simulink model "Model_LQR_Ideal"  (R2025a)
settings: Solver=ode4  StartTime=0.0  StopTime=inf  FixedStep=0.0001  RelTol=1e-3
InitFcn:
  | addpath('functions');
model workspace: external: MATLAB File D:\OneDrive - University of Bristol\2025-2026\grp-major_project - General\LQR\furuta-inverted-pendulum-LQR\init_LQR.m (data not in the file)
values from neighbouring files (symbols this model uses):
  I_1 = in2(:,4)    [furuta_single_A_B_matrices.m]    (also in furuta_single_state_derivative.m = in4(:,4); init_LQR.m = 0.00011)
  I_arm = in2(:,2)    [furuta_single_A_B_matrices.m]    (also in furuta_single_state_derivative.m = in4(:,2); init_LQR.m = 0.000739)
  init_S = [0; 0; 0.26; 0]    [init_LQR.m]
  K = lqr(A, B, Q, R)    [init_LQR.m]
  L_1 = 0.14    [init_LQR.m]    (also in playback_animation_single.m = out.plotData.L_1.Data(1))
  L_arm = in2(:,1)    [furuta_single_A_B_matrices.m]    (also in furuta_single_state_derivative.m = in4(:,1); init_LQR.m = 0.1475; playback_animation_single.m = out.plotData.L_arm.Data(1))
  lcom_1 = in2(:,3)    [furuta_single_A_B_matrices.m]    (also in furuta_single_state_derivative.m = in4(:,3); init_LQR.m = 0.051; playback_animation_single.m = out.plotData.lcom_1.Data(1))
  m_1 = in2(:,5)    [furuta_single_A_B_matrices.m]    (also in furuta_single_state_derivative.m = in4(:,5); init_LQR.m = 0.054)
settings Model: PacingRate=0.010000  Creator=Esther  LastModifiedBy=Hankin

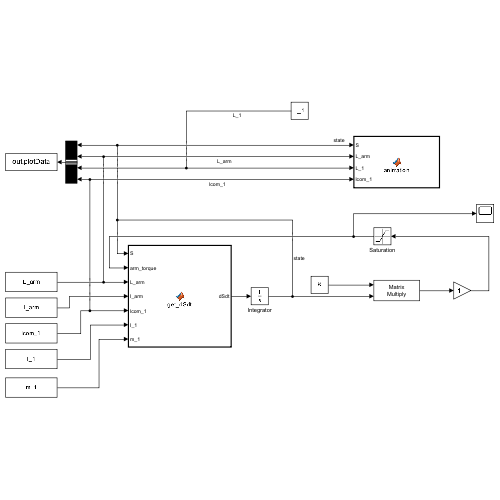
[thumbnail: Simulink's stored preview of the top-level diagram]
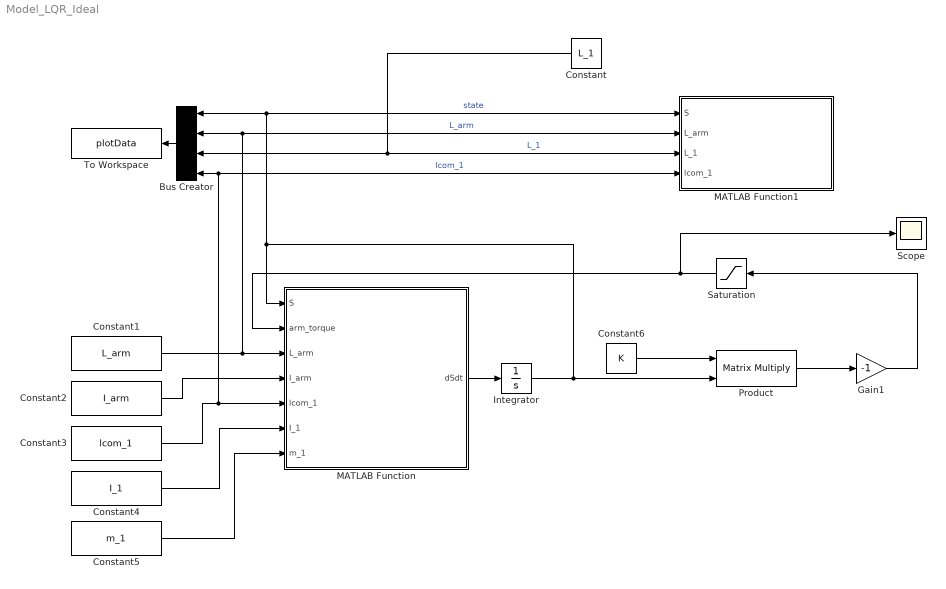
== system Model_LQR_Ideal ==
  Bus Creator : BusCreator  Inputs=4
  Constant : Constant  Value=L_1
  Constant1 : Constant  Value=L_arm
  Constant2 : Constant  Value=I_arm
  Constant3 : Constant  Value=lcom_1
  Constant4 : Constant  Value=I_1
  Constant5 : Constant  Value=m_1
  Constant6 : Constant  Value=K  VectorParams1D=off
  Gain1 : Gain  Gain=-1
  Integrator : Integrator  InitialCondition=init_S
  MATLAB Function : MATLAB Function  TreatAsAtomicUnit=on
  MATLAB Function1 : MATLAB Function  TreatAsAtomicUnit=on
  Product : Product  Multiplication=Matrix(*)
  Saturation : Saturate  UpperLimit=0.088  LowerLimit=-0.088
  Scope : Scope
      settings: ActiveDisplayYMinimum=-0.10999999999999999  ActiveDisplayYMaximum=0.10999999999999999
  To Workspace : ToWorkspace  VariableName=plotData  SaveFormat=Timeseries  SampleTime=-1
  wires:
  MATLAB Function/1(dSdt) -> Integrator/1
  Constant1/1 -> MATLAB Function/3(L_arm), Bus Creator/2, MATLAB Function1/2(L_arm)  "L_arm"
  Constant2/1 -> MATLAB Function/4(I_arm)
  Constant3/1 -> MATLAB Function/5(lcom_1), Bus Creator/4, MATLAB Function1/4(lcom_1)  "lcom_1"
  Constant4/1 -> MATLAB Function/6(I_1)
  Constant5/1 -> MATLAB Function/7(m_1)
  Integrator/1 -> MATLAB Function/1(S), Bus Creator/1, MATLAB Function1/1(S), Product/2  "state"
  Bus Creator/1 -> To Workspace/1
  Constant/1 -> MATLAB Function1/3(L_1), Bus Creator/3  "L_1"
  Product/1 -> Gain1/1
  Constant6/1 -> Product/1
  Saturation/1 -> Scope/1, MATLAB Function/2(arm_torque)
  Gain1/1 -> Saturation/1

== matlab function Model_LQR_Ideal/MATLAB Function1 ==
  settings: updateMethod=DISCRETE
  data: S input; L_arm input; L_1 input; lcom_1 input
function animation(S, L_arm, L_1, lcom_1)
    update_ratio = 100;
    realtime_animation_single(S, L_arm, L_1, lcom_1, update_ratio);
end

== matlab function Model_LQR_Ideal/MATLAB Function ==
  data: S input size=4; dSdt output size=4; arm_torque input size=1; L_arm input size=1; I_arm input size=1; lcom_1 input size=1; I_1 input size=1; m_1 input size=1
function dSdt = get_dSdt(S, arm_torque, L_arm, I_arm, lcom_1, I_1, m_1)
    t = 0;
    g = 9.81;
    phys_param = [L_arm, I_arm, lcom_1, I_1, m_1, g];
    fric_arm = [0.0034, 0.01, 100];
    fric_1 = [0.001, 0.0001, 100];
    dSdt = furuta_single_state_derivative(t, S, arm_torque, phys_param, fric_arm, fric_1);
end
